simulink library "AntiRollBar_Droplink_Rod"  (R2025a)
settings: Solver=VariableStepAuto  StartTime=0.0  StopTime=10.0  RelTol=1e-3
undefined symbols (not defined in the file): AntiRollBar, Visual, X, Y, Z
libraries: sm_lib x15, Suspension_Utilities x9, nesl_utility x1
Description:
  | Component of Simscape Vehicle Templates Library
  | 
  | Copyright 2018-2026 The MathWorks, Inc.
settings Model: Creator=smiller  LastModifiedBy=smiller
settings SolverCC: AlgebraicLoopSolver=TrustRegion
settings DataIOCC: ReturnWorkspaceOutputs=off
settings OptimizationCC: ReuseModelBlockBuffer=off
settings DebuggingCC: UnconnectedInputMsg=warning  UnconnectedOutputMsg=warning  UnconnectedLineMsg=warning  ArithmeticOperatorsInVariantConditions=warning
settings ModelReferenceCC: EnableRefExpFcnMdlSchedulingChecks=on
settings SFSimCC: CustomCodeUndefinedFunction=UseInterfaceOnly
settings RTWCC: GPUComputeCapability=3.5  DLArmComputeVersion=19.05

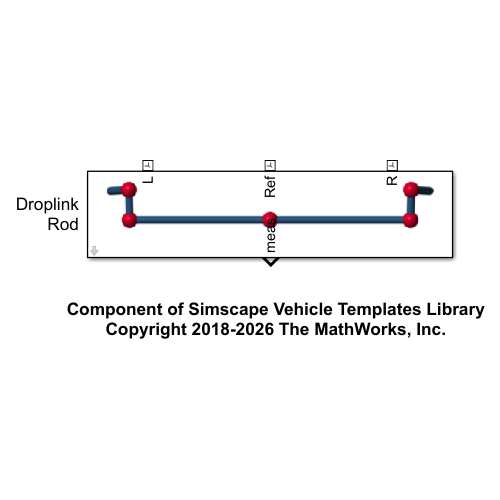
[thumbnail: Simulink's stored preview of the top-level diagram]
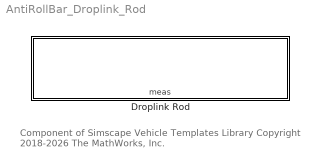
== system AntiRollBar_Droplink_Rod ==
  note: Component of Simscape Vehicle Templates Library
      | Copyright 2018-2026 The MathWorks, Inc.
  Droplink Rod : Subsystem  VariantControl=DroplinkRod  mask(Anti-Roll Bar with Droplink Connection){hp_rod=AntiRollBar.sSuspension.Value, hp_out=AntiRollBar.sOutboard.Value, hp_in=AntiRollBar.sInboard.Value, hp_mount_subframe=AntiRollBar.sMount.Value, rotYAxis=AntiRollBar.qUniversal.Value, SubframeConnection=AntiRollBar.SubframeConnection, k=AntiRollBar.k.Value, d=AntiRollBar.d.Value, m=AntiRollBar.m.Value, clr_solid=Visual.AntiRollBar.clr, opc_solid=Visual.part.opc, rad_solid=Visual.AntiRollBar.rad, clr_hp=Visual.hp.clr, opc_hp=Visual.hp.opc, rad_hp=Visual.hp.rad}
      mask prompts: hp_rod "HP Rod to Suspension [xyz] (m)"; hp_out "HP Outboard [xyz] (m)"; hp_in "HP Inboard [xyz] (m)"; hp_mount_subframe "HP Mount Subframe [xyz] (m)"; rotYAxis "Universal Joint Y Rotation (deg)"; SubframeConnection "Subframe Connection"; k "Stiffness (N*m/(deg))"; d "Damping (N*m/(deg/s))"; m "Mass"
      mask help: Models anti-roll bar with drop link connection to left and right suspension.
      mask TypeOptions rotYAxis:
      | Universal
      | Rod SuspL/rotYAxis | Universal
      | Rod SuspR/rotYAxis
      mask TypeOptions clr_solid:
      | ARB Left/clr_solid | ARB Right/clr_solid | Lever
      | Left/clr_solid | Lever
      | Right/clr_solid
      mask TypeOptions opc_solid:
      | ARB Left/opc_solid | ARB Right/opc_solid | Lever
      | Left/opc_solid | Lever
      | Right/opc_solid
      mask TypeOptions rad_solid:
      | ARB Left/rad_solid | ARB Right/rad_solid | Lever
      | Left/rad_solid | Lever
      | Right/rad_solid
      mask TypeOptions clr_hp:
      | Vis HP
      | ARB Flex/GraphicDiffuseColor | Vis HP
      | ARB Out L/GraphicDiffuseColor | Vis HP
      | ARB Out R/GraphicDiffuseColor | Vis HP
      | ARB In L/GraphicDiffuseColor | Vis HP
      | ARB In R/GraphicDiffuseColor
      mask TypeOptions opc_hp:
      | Vis HP
      | ARB Flex/GraphicOpacity | Vis HP
      | ARB Out L/GraphicOpacity | Vis HP
      | ARB Out R/GraphicOpacity | Vis HP
      | ARB In L/GraphicOpacity | Vis HP
      | ARB In R/GraphicOpacity
      mask TypeOptions rad_hp:
      | Vis HP
      | ARB Flex/SphereRadius | Vis HP
      | ARB Out L/SphereRadius | Vis HP
      | ARB Out R/SphereRadius | Vis HP
      | ARB In L/SphereRadius | Vis HP
      | ARB In R/SphereRadius
      mask DialogControl cont_vis Prompt: Visualization
      mask DialogControl text_vis_clr Prompt: Color [RGB]
      mask DialogControl text_vis_opc Prompt: Opacity (0-1)
      mask DialogControl text_vis_size Prompt: Size (m)
      mask DialogControl text_vis_bar Prompt: Bar
      mask DialogControl text_vis_hardpoints Prompt: Hardpoints
      mask Display: image('sm_car_vehicle_linkage_antirollbar_rod_IMAGE.png');

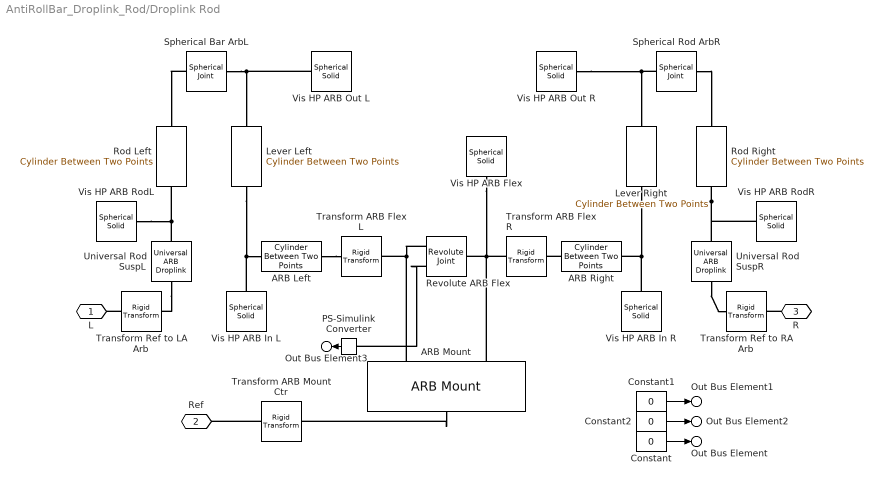
== system AntiRollBar_Droplink_Rod/Droplink Rod ==
  ARB Left : Suspension_Utilities/Cylinder Between Two Points  hp_b=hp_in.*[1 0 1]  hp_f=hp_in  Mass=m/4  clr_solid=clr_solid  opc_solid=opc_solid  rad_solid=rad_solid
  ARB Mount : Suspension_Utilities/ARB Mount  VariantControl=Choice  LabelModeActiveChoice=Rigid_1Rev  Connection=SubframeConnection  VariantLabel=SubframeConnection.class.Value
      settings: AttributesFormatString=%<LabelModeActiveChoice>
  ARB Right : Suspension_Utilities/Cylinder Between Two Points  hp_b=hp_in.*[1 -1 1]  hp_f=hp_in.*[1 0 1]  Mass=m/4  clr_solid=clr_solid  opc_solid=opc_solid  rad_solid=rad_solid
  Constant : Constant  Value=0
  Constant1 : Constant  Value=0
  Constant2 : Constant  Value=0
  Lever Left : Suspension_Utilities/Cylinder Between Two Points  hp_b=hp_in  hp_f=hp_out  Mass=m/4  clr_solid=clr_solid  opc_solid=opc_solid  rad_solid=rad_solid
  Lever Right : Suspension_Utilities/Cylinder Between Two Points  hp_b=hp_out.*[1 -1 1]  hp_f=hp_in.*[1 -1 1]  Mass=m/4  clr_solid=clr_solid  opc_solid=opc_solid  rad_solid=rad_solid
  PS-Simulink Converter : nesl_utility/PS-Simulink Converter  PhysicalDomain=network_engine_domain  SubClassName=ps_output  LeftPortType=input  RightPortType=output  PseudoPeriodic=off  Frequencies=[]  VectorFormat=1-D array  Unit=1  AffineConversion=off
  Revolute ARB Flex : sm_lib/Joints/Revolute Joint  JointMode=Normal  CompositeWrenchDir=FollowerOnBase  CompositeWrenchFrame=BaseFrame  SenseConstraintForce=off  SenseConstraintTorque=off  SenseTotalForce=off  SenseTotalTorque=off  PositionTargetSpecify=on  PositionTargetPriority=Low  PositionTargetValue=0  PositionTargetValueUnits=deg  VelocityTargetSpecify=off  VelocityTargetPriority=High  VelocityTargetValue=0  VelocityTargetValueUnits=deg/s  EquilibriumPosition=0  EquilibriumPositionUnits=deg  SpringStiffness=k  SpringStiffnessUnits=N*m/deg  DampingCoefficient=d  DampingCoefficientUnits=N*m/(deg/s)  LowerLimitSpecify=off  LowerLimitBound=-90  LowerLimitBoundUnits=deg  LowerLimitStiffness=1e4  LowerLimitStiffnessUnits=N*m/deg  LowerLimitDamping=10  LowerLimitDampingUnits=N*m/(deg/s)  LowerLimitTransitionRegionWidth=0.1  LowerLimitTransitionRegionWidthUnits=deg  UpperLimitSpecify=off  UpperLimitBound=90  UpperLimitBoundUnits=deg  UpperLimitStiffness=1e4  UpperLimitStiffnessUnits=N*m/deg  UpperLimitDamping=10  UpperLimitDampingUnits=N*m/(deg/s)  UpperLimitTransitionRegionWidth=0.1  UpperLimitTransitionRegionWidthUnits=deg  TorqueActuationMode=NoTorque  MotionActuationMode=ComputedMotion  SensePosition=on  SenseVelocity=off  SenseAcceleration=off  SenseTorqueForce=off  SenseLowerLimitTorqueForce=off  SenseUpperLimitTorqueForce=off
  Rod Left : Suspension_Utilities/Cylinder Between Two Points  hp_b=hp_out  hp_f=hp_rod  Mass=m/4  clr_solid=clr_solid  opc_solid=opc_solid  rad_solid=rad_solid
  Rod Right : Suspension_Utilities/Cylinder Between Two Points  hp_b=hp_rod.*[1 -1 1]  hp_f=hp_out.*[1 -1 1]  Mass=m/4  clr_solid=clr_solid  opc_solid=opc_solid  rad_solid=rad_solid
  Spherical Bar ArbL : sm_lib/Joints/Spherical Joint  JointMode=Normal  CompositeWrenchDir=FollowerOnBase  CompositeWrenchFrame=BaseFrame  SenseConstraintForce=off  SenseConstraintTorque=off  SenseTotalForce=off  SenseTotalTorque=off  PositionTargetSpecify=off  PositionTargetPriority=High  PositionTargetRotationMethod=None  PositionTargetFollAlignAxisA=+X  PositionTargetBaseAlignAxisA=+Y  PositionTargetFollAlignAxisB=+Y  PositionTargetBaseAlignAxisB=+Z  PositionTargetRotationStandardAxis=+Z  PositionTargetRotationAngle=0.0  PositionTargetRotationAngleUnits=deg  PositionTargetRotationArbitraryAxis=[0 0 1]  PositionTargetRotationSequenceAxes=FollowerAxes  PositionTargetRotationSequence=XYX  PositionTargetRotationSequenceAngles=[0 0 0]  PositionTargetRotationSequenceAnglesUnits=deg  PositionTargetRotationMatrix=[1 0 0; 0 1 0; 0 0 1]  PositionTargetQuaternion=[1 0 0 0]  VelocityTargetSpecify=off  VelocityTargetPriority=High  VelocityTargetValue=[0 0 0]  VelocityTargetValueUnits=deg/s  VelocityTargetInFollowerFrame=on  EqPosRotationMethod=None  EqPosFollAlignAxisA=+X  EqPosBaseAlignAxisA=+Y  EqPosFollAlignAxisB=+Y  EqPosBaseAlignAxisB=+Z  EqPosRotationStandardAxis=+Z  EqPosRotationAngle=0.0  EqPosRotationAngleUnits=deg  EqPosRotationArbitraryAxis=[0 0 1]  EqPosRotationSequenceAxes=FollowerAxes  EqPosRotationSequence=XYX  EqPosRotationSequenceAngles=[0 0 0]  EqPosRotationSequenceAnglesUnits=deg  EqPosRotationMatrix=[1 0 0; 0 1 0; 0 0 1]  EqPosQuaternion=[1 0 0 0]  SpringStiffness=0  SpringStiffnessUnits=N*m/deg  DampingCoefficient=0  DampingCoefficientUnits=N*m/(deg/s)  LowerLimitSpecify=off  LowerLimitBound=15  LowerLimitBoundUnits=deg  LowerLimitStiffness=1e4  LowerLimitStiffnessUnits=N*m/deg  LowerLimitDamping=10  LowerLimitDampingUnits=N*m/(deg/s)  LowerLimitTransitionRegionWidth=0.1  LowerLimitTransitionRegionWidthUnits=deg  UpperLimitSpecify=off  UpperLimitBound=45  UpperLimitBoundUnits=deg  UpperLimitStiffness=1e4  UpperLimitStiffnessUnits=N*m/deg  UpperLimitDamping=10  UpperLimitDampingUnits=N*m/(deg/s)  UpperLimitTransitionRegionWidth=0.1  UpperLimitTransitionRegionWidthUnits=deg  TorqueActuationMode=NoTorque  ActuateTorqueX=off  ActuateTorqueY=off  ActuateTorqueZ=off  ActuateTorque=off  ActuationFrame=BaseFrame  SensePosition=off  SenseVelocityX=off  SenseVelocityY=off  SenseVelocityZ=off  SenseVelocity=off  SenseAccelerationX=off  SenseAccelerationY=off  SenseAccelerationZ=off  SenseAcceleration=off  SenseLowerLimitTorqueMag=off  SenseUpperLimitTorqueMag=off  SensingFrame=BaseFrame
  Spherical Rod ArbR : sm_lib/Joints/Spherical Joint  JointMode=Normal  CompositeWrenchDir=FollowerOnBase  CompositeWrenchFrame=BaseFrame  SenseConstraintForce=off  SenseConstraintTorque=off  SenseTotalForce=off  SenseTotalTorque=off  PositionTargetSpecify=off  PositionTargetPriority=High  PositionTargetRotationMethod=None  PositionTargetFollAlignAxisA=+X  PositionTargetBaseAlignAxisA=+Y  PositionTargetFollAlignAxisB=+Y  PositionTargetBaseAlignAxisB=+Z  PositionTargetRotationStandardAxis=+Z  PositionTargetRotationAngle=0.0  PositionTargetRotationAngleUnits=deg  PositionTargetRotationArbitraryAxis=[0 0 1]  PositionTargetRotationSequenceAxes=FollowerAxes  PositionTargetRotationSequence=XYX  PositionTargetRotationSequenceAngles=[0 0 0]  PositionTargetRotationSequenceAnglesUnits=deg  PositionTargetRotationMatrix=[1 0 0; 0 1 0; 0 0 1]  PositionTargetQuaternion=[1 0 0 0]  VelocityTargetSpecify=off  VelocityTargetPriority=High  VelocityTargetValue=[0 0 0]  VelocityTargetValueUnits=deg/s  VelocityTargetInFollowerFrame=on  EqPosRotationMethod=None  EqPosFollAlignAxisA=+X  EqPosBaseAlignAxisA=+Y  EqPosFollAlignAxisB=+Y  EqPosBaseAlignAxisB=+Z  EqPosRotationStandardAxis=+Z  EqPosRotationAngle=0.0  EqPosRotationAngleUnits=deg  EqPosRotationArbitraryAxis=[0 0 1]  EqPosRotationSequenceAxes=FollowerAxes  EqPosRotationSequence=XYX  EqPosRotationSequenceAngles=[0 0 0]  EqPosRotationSequenceAnglesUnits=deg  EqPosRotationMatrix=[1 0 0; 0 1 0; 0 0 1]  EqPosQuaternion=[1 0 0 0]  SpringStiffness=0  SpringStiffnessUnits=N*m/deg  DampingCoefficient=0  DampingCoefficientUnits=N*m/(deg/s)  LowerLimitSpecify=off  LowerLimitBound=15  LowerLimitBoundUnits=deg  LowerLimitStiffness=1e4  LowerLimitStiffnessUnits=N*m/deg  LowerLimitDamping=10  LowerLimitDampingUnits=N*m/(deg/s)  LowerLimitTransitionRegionWidth=0.1  LowerLimitTransitionRegionWidthUnits=deg  UpperLimitSpecify=off  UpperLimitBound=45  UpperLimitBoundUnits=deg  UpperLimitStiffness=1e4  UpperLimitStiffnessUnits=N*m/deg  UpperLimitDamping=10  UpperLimitDampingUnits=N*m/(deg/s)  UpperLimitTransitionRegionWidth=0.1  UpperLimitTransitionRegionWidthUnits=deg  TorqueActuationMode=NoTorque  ActuateTorqueX=off  ActuateTorqueY=off  ActuateTorqueZ=off  ActuateTorque=off  ActuationFrame=BaseFrame  SensePosition=off  SenseVelocityX=off  SenseVelocityY=off  SenseVelocityZ=off  SenseVelocity=off  SenseAccelerationX=off  SenseAccelerationY=off  SenseAccelerationZ=off  SenseAcceleration=off  SenseLowerLimitTorqueMag=off  SenseUpperLimitTorqueMag=off  SensingFrame=BaseFrame
  Transform ARB Flex L : sm_lib/Frames and Transforms/Rigid Transform  RotationMethod=StandardAxis  FollAlignAxisA=+X  BaseAlignAxisA=+Y  FollAlignAxisB=+Y  BaseAlignAxisB=+Z  RotationStandardAxis=+X  RotationAngle=-90  RotationAngleUnits=deg  RotationArbitraryAxis=[0 0 1]  RotationSequenceAxes=FollowerAxes  RotationSequence=XYX  RotationSequenceAngles=[0 0 0]  RotationSequenceAnglesUnits=deg  RotationMatrix=[1 0 0; 0 1 0; 0 0 1]  Quaternion=[1 0 0 0]  TranslationMethod=None  TranslationCartesianOffset=[0 0 0]  TranslationCartesianOffsetUnits=m  TranslationStandardAxis=+Z  TranslationStandardOffset=0  TranslationStandardOffsetUnits=m  TranslationROffset=0  TranslationROffsetUnits=m  TranslationThetaOffset=0  TranslationThetaOffsetUnits=deg  TranslationZOffset=0  TranslationZOffsetUnits=m
  Transform ARB Flex R : sm_lib/Frames and Transforms/Rigid Transform  RotationMethod=StandardAxis  FollAlignAxisA=+X  BaseAlignAxisA=+Y  FollAlignAxisB=+Y  BaseAlignAxisB=+Z  RotationStandardAxis=+X  RotationAngle=-90  RotationAngleUnits=deg  RotationArbitraryAxis=[0 0 1]  RotationSequenceAxes=FollowerAxes  RotationSequence=XYX  RotationSequenceAngles=[0 0 0]  RotationSequenceAnglesUnits=deg  RotationMatrix=[1 0 0; 0 1 0; 0 0 1]  Quaternion=[1 0 0 0]  TranslationMethod=None  TranslationCartesianOffset=[0 0 0]  TranslationCartesianOffsetUnits=m  TranslationStandardAxis=+Z  TranslationStandardOffset=0  TranslationStandardOffsetUnits=m  TranslationROffset=0  TranslationROffsetUnits=m  TranslationThetaOffset=0  TranslationThetaOffsetUnits=deg  TranslationZOffset=0  TranslationZOffsetUnits=m
  Transform ARB Mount Ctr : sm_lib/Frames and Transforms/Rigid Transform  RotationMethod=StandardAxis  FollAlignAxisA=+X  BaseAlignAxisA=+Y  FollAlignAxisB=+Y  BaseAlignAxisB=+Z  RotationStandardAxis=+X  RotationAngle=-90  RotationAngleUnits=deg  RotationArbitraryAxis=[0 0 1]  RotationSequenceAxes=FollowerAxes  RotationSequence=XYX  RotationSequenceAngles=[0 0 0]  RotationSequenceAnglesUnits=deg  RotationMatrix=[1 0 0; 0 1 0; 0 0 1]  Quaternion=[1 0 0 0]  TranslationMethod=Cartesian  TranslationCartesianOffset=hp_in.*[1 0 1]  TranslationCartesianOffsetUnits=m  TranslationStandardAxis=+Z  TranslationStandardOffset=0  TranslationStandardOffsetUnits=m  TranslationROffset=0  TranslationROffsetUnits=m  TranslationThetaOffset=0  TranslationThetaOffsetUnits=deg  TranslationZOffset=0  TranslationZOffsetUnits=m
  Transform Ref to LA Arb : sm_lib/Frames and Transforms/Rigid Transform  RotationMethod=None  FollAlignAxisA=+X  BaseAlignAxisA=+Y  FollAlignAxisB=+Y  BaseAlignAxisB=+Z  RotationStandardAxis=+Z  RotationAngle=0.0  RotationAngleUnits=deg  RotationArbitraryAxis=[0 0 1]  RotationSequenceAxes=FollowerAxes  RotationSequence=XYX  RotationSequenceAngles=[0 0 0]  RotationSequenceAnglesUnits=deg  RotationMatrix=[1 0 0; 0 1 0; 0 0 1]  Quaternion=[1 0 0 0]  TranslationMethod=Cartesian  TranslationCartesianOffset=hp_rod  TranslationCartesianOffsetUnits=m  TranslationStandardAxis=+Z  TranslationStandardOffset=0  TranslationStandardOffsetUnits=m  TranslationROffset=0  TranslationROffsetUnits=m  TranslationThetaOffset=0  TranslationThetaOffsetUnits=deg  TranslationZOffset=0  TranslationZOffsetUnits=m
  Transform Ref to RA Arb : sm_lib/Frames and Transforms/Rigid Transform  RotationMethod=None  FollAlignAxisA=+X  BaseAlignAxisA=+Y  FollAlignAxisB=+Y  BaseAlignAxisB=+Z  RotationStandardAxis=+Z  RotationAngle=0.0  RotationAngleUnits=deg  RotationArbitraryAxis=[0 0 1]  RotationSequenceAxes=FollowerAxes  RotationSequence=XYX  RotationSequenceAngles=[0 0 0]  RotationSequenceAnglesUnits=deg  RotationMatrix=[1 0 0; 0 1 0; 0 0 1]  Quaternion=[1 0 0 0]  TranslationMethod=Cartesian  TranslationCartesianOffset=hp_rod.*[1 -1 1]  TranslationCartesianOffsetUnits=m  TranslationStandardAxis=+Z  TranslationStandardOffset=0  TranslationStandardOffsetUnits=m  TranslationROffset=0  TranslationROffsetUnits=m  TranslationThetaOffset=0  TranslationThetaOffsetUnits=deg  TranslationZOffset=0  TranslationZOffsetUnits=m
  Universal Rod SuspL : Suspension_Utilities/Universal ARB Droplink  rotYAxis=rotYAxis
  Universal Rod SuspR : Suspension_Utilities/Universal ARB Droplink  rotYAxis=rotYAxis
  Vis HP ARB Flex : sm_lib/Body Elements/Spherical Solid  SphereRadius=rad_hp  SphereRadiusUnits=m  ExportEntireGeometry=off  InertiaType=CalculateFromGeometry  BasedOnType=Density  Density=1000  DensityUnits=kg/m^3  Mass=1  MassUnits=kg  CenterOfMass=[0 0 0]  CenterOfMassUnits=m  MomentsOfInertia=[1 1 1]  MomentsOfInertiaUnits=kg*m^2  ProductsOfInertia=[0 0 0]  ProductsOfInertiaUnits=kg*m^2  GraphicType=FromGeometry  MarkerShape=Sphere  MarkerSize=10  GraphicVisPropType=SimpleVisualProperties  GraphicDiffuseColor=clr_hp  GraphicOpacity=opc_hp  GraphicSpecularColor=[0.5 0.5 0.5 1.0]  GraphicAmbientColor=[0.15 0.15 0.15 1.0]  GraphicEmissiveColor=[0.0 0.0 0.0 1.0]  GraphicShininess=75  DoExposeReferenceFrame=on  SerializedFrames=<Frames/>
  Vis HP ARB In L : sm_lib/Body Elements/Spherical Solid  SphereRadius=rad_hp  SphereRadiusUnits=m  ExportEntireGeometry=off  InertiaType=CalculateFromGeometry  BasedOnType=Density  Density=1000  DensityUnits=kg/m^3  Mass=1  MassUnits=kg  CenterOfMass=[0 0 0]  CenterOfMassUnits=m  MomentsOfInertia=[1 1 1]  MomentsOfInertiaUnits=kg*m^2  ProductsOfInertia=[0 0 0]  ProductsOfInertiaUnits=kg*m^2  GraphicType=FromGeometry  MarkerShape=Sphere  MarkerSize=10  GraphicVisPropType=SimpleVisualProperties  GraphicDiffuseColor=clr_hp  GraphicOpacity=opc_hp  GraphicSpecularColor=[0.5 0.5 0.5 1.0]  GraphicAmbientColor=[0.15 0.15 0.15 1.0]  GraphicEmissiveColor=[0.0 0.0 0.0 1.0]  GraphicShininess=75  DoExposeReferenceFrame=on  SerializedFrames=<Frames/>
  Vis HP ARB In R : sm_lib/Body Elements/Spherical Solid  SphereRadius=rad_hp  SphereRadiusUnits=m  ExportEntireGeometry=off  InertiaType=CalculateFromGeometry  BasedOnType=Density  Density=1000  DensityUnits=kg/m^3  Mass=1  MassUnits=kg  CenterOfMass=[0 0 0]  CenterOfMassUnits=m  MomentsOfInertia=[1 1 1]  MomentsOfInertiaUnits=kg*m^2  ProductsOfInertia=[0 0 0]  ProductsOfInertiaUnits=kg*m^2  GraphicType=FromGeometry  MarkerShape=Sphere  MarkerSize=10  GraphicVisPropType=SimpleVisualProperties  GraphicDiffuseColor=clr_hp  GraphicOpacity=opc_hp  GraphicSpecularColor=[0.5 0.5 0.5 1.0]  GraphicAmbientColor=[0.15 0.15 0.15 1.0]  GraphicEmissiveColor=[0.0 0.0 0.0 1.0]  GraphicShininess=75  DoExposeReferenceFrame=on  SerializedFrames=<Frames/>
  Vis HP ARB Out L : sm_lib/Body Elements/Spherical Solid  SphereRadius=rad_hp  SphereRadiusUnits=m  ExportEntireGeometry=off  InertiaType=CalculateFromGeometry  BasedOnType=Density  Density=1000  DensityUnits=kg/m^3  Mass=1  MassUnits=kg  CenterOfMass=[0 0 0]  CenterOfMassUnits=m  MomentsOfInertia=[1 1 1]  MomentsOfInertiaUnits=kg*m^2  ProductsOfInertia=[0 0 0]  ProductsOfInertiaUnits=kg*m^2  GraphicType=FromGeometry  MarkerShape=Sphere  MarkerSize=10  GraphicVisPropType=SimpleVisualProperties  GraphicDiffuseColor=clr_hp  GraphicOpacity=opc_hp  GraphicSpecularColor=[0.5 0.5 0.5 1.0]  GraphicAmbientColor=[0.15 0.15 0.15 1.0]  GraphicEmissiveColor=[0.0 0.0 0.0 1.0]  GraphicShininess=75  DoExposeReferenceFrame=on  SerializedFrames=<Frames/>
  Vis HP ARB Out R : sm_lib/Body Elements/Spherical Solid  SphereRadius=rad_hp  SphereRadiusUnits=m  ExportEntireGeometry=off  InertiaType=CalculateFromGeometry  BasedOnType=Density  Density=1000  DensityUnits=kg/m^3  Mass=1  MassUnits=kg  CenterOfMass=[0 0 0]  CenterOfMassUnits=m  MomentsOfInertia=[1 1 1]  MomentsOfInertiaUnits=kg*m^2  ProductsOfInertia=[0 0 0]  ProductsOfInertiaUnits=kg*m^2  GraphicType=FromGeometry  MarkerShape=Sphere  MarkerSize=10  GraphicVisPropType=SimpleVisualProperties  GraphicDiffuseColor=clr_hp  GraphicOpacity=opc_hp  GraphicSpecularColor=[0.5 0.5 0.5 1.0]  GraphicAmbientColor=[0.15 0.15 0.15 1.0]  GraphicEmissiveColor=[0.0 0.0 0.0 1.0]  GraphicShininess=75  DoExposeReferenceFrame=on  SerializedFrames=<Frames/>
  Vis HP ARB RodL : sm_lib/Body Elements/Spherical Solid  SphereRadius=rad_hp  SphereRadiusUnits=m  ExportEntireGeometry=off  InertiaType=CalculateFromGeometry  BasedOnType=Density  Density=1000  DensityUnits=kg/m^3  Mass=1  MassUnits=kg  CenterOfMass=[0 0 0]  CenterOfMassUnits=m  MomentsOfInertia=[1 1 1]  MomentsOfInertiaUnits=kg*m^2  ProductsOfInertia=[0 0 0]  ProductsOfInertiaUnits=kg*m^2  GraphicType=FromGeometry  MarkerShape=Sphere  MarkerSize=10  GraphicVisPropType=SimpleVisualProperties  GraphicDiffuseColor=clr_hp  GraphicOpacity=opc_hp  GraphicSpecularColor=[0.5 0.5 0.5 1.0]  GraphicAmbientColor=[0.15 0.15 0.15 1.0]  GraphicEmissiveColor=[0.0 0.0 0.0 1.0]  GraphicShininess=75  DoExposeReferenceFrame=on  SerializedFrames=<Frames/>
  Vis HP ARB RodR : sm_lib/Body Elements/Spherical Solid  SphereRadius=rad_hp  SphereRadiusUnits=m  ExportEntireGeometry=off  InertiaType=CalculateFromGeometry  BasedOnType=Density  Density=1000  DensityUnits=kg/m^3  Mass=1  MassUnits=kg  CenterOfMass=[0 0 0]  CenterOfMassUnits=m  MomentsOfInertia=[1 1 1]  MomentsOfInertiaUnits=kg*m^2  ProductsOfInertia=[0 0 0]  ProductsOfInertiaUnits=kg*m^2  GraphicType=FromGeometry  MarkerShape=Sphere  MarkerSize=10  GraphicVisPropType=SimpleVisualProperties  GraphicDiffuseColor=clr_hp  GraphicOpacity=opc_hp  GraphicSpecularColor=[0.5 0.5 0.5 1.0]  GraphicAmbientColor=[0.15 0.15 0.15 1.0]  GraphicEmissiveColor=[0.0 0.0 0.0 1.0]  GraphicShininess=75  DoExposeReferenceFrame=on  SerializedFrames=<Frames/>
  L : PMIOPort  Side=Left
  Ref : PMIOPort  Port=2  Side=Left
  R : PMIOPort  Port=3  Side=Left
  Out Bus Element : Outport  VectorParamsAs1DForOutWhenUnconnected=off  PortName=meas  Element=zLA
  Out Bus Element1 : Outport  VectorParamsAs1DForOutWhenUnconnected=off  PortName=meas  Element=zRA
  Out Bus Element2 : Outport  VectorParamsAs1DForOutWhenUnconnected=off  PortName=meas  Element=fARB
  Out Bus Element3 : Outport  VectorParamsAs1DForOutWhenUnconnected=off  PortName=meas  Element=q
  wires:
  Constant2/1 -> Out Bus Element2/1
  Constant1/1 -> Out Bus Element1/1
  Constant/1 -> Out Bus Element/1
  PS-Simulink Converter/1 -> Out Bus Element3/1
  connections:
  Transform ARB Mount Ctr/LConn1 -- Ref/RConn1
  Transform Ref to LA Arb/LConn1 -- L/RConn1
  R/RConn1 -- Transform Ref to RA Arb/LConn1
  Vis HP ARB Out L/RConn1 -- Spherical Bar ArbL/LConn1 -- Lever Left/RConn1
  Revolute ARB Flex/RConn1 -- ARB Mount/RConn1 -- Transform ARB Flex L/RConn1
  Vis HP ARB In L/RConn1 -- Lever Left/LConn1 -- ARB Left/RConn1
  ARB Mount/RConn2 -- Vis HP ARB Flex/RConn1 -- Revolute ARB Flex/LConn1 -- Transform ARB Flex R/RConn1
  Vis HP ARB In R/RConn1 -- Lever Right/RConn1 -- ARB Right/LConn1
  Vis HP ARB Out R/RConn1 -- Spherical Rod ArbR/RConn1 -- Lever Right/LConn1
  ARB Right/RConn1 -- Transform ARB Flex R/LConn1
  ARB Left/LConn1 -- Transform ARB Flex L/LConn1
  Revolute ARB Flex/RConn2 -- PS-Simulink Converter/LConn1
  Spherical Rod ArbR/LConn1 -- Rod Right/RConn1
  Spherical Bar ArbL/RConn1 -- Rod Left/LConn1
  ARB Mount/LConn1 -- Transform ARB Mount Ctr/RConn1
  Vis HP ARB RodL/RConn1 -- Universal Rod SuspL/LConn1 -- Rod Left/RConn1
  Universal Rod SuspL/RConn1 -- Transform Ref to LA Arb/RConn1
  Rod Right/LConn1 -- Universal Rod SuspR/LConn1 -- Vis HP ARB RodR/RConn1
  Universal Rod SuspR/RConn1 -- Transform Ref to RA Arb/RConn1
